simulink model "commqpsktxrx_18b"  (R2018b)
settings: Solver=FixedStepDiscrete  StartTime=0.0  StopTime=inf  RelTol=1e-3
PreLoadFcn:
  | qpsktxrx = commqpsktxrx_init();
InitFcn:
  | qpsktxrx = commqpsktxrx_init();
StopFcn:
  | if (strcmp(get_param([bdroot, '/Model Parameters'],'ShowRecvMsg'),'on'))
  |   if exist('Received','var')
  |      fprintf('%s', Received.signals.values);
  |   end
  | end
undefined symbols (not defined in the file or in its folder): Fs, ip, usb
libraries: dspsigops x3, commdigbbndpm3 x3, commsync2 x3, plutoradiolib x2, simulink x2, commrflib2 x2, commrfcorlib x2, dspstat3 x2, commutil2 x2, commsequence2 x2, dspsrcs4 x2, commfilt2 x2
Description:
  | QPSK Transmitter and Receiver.
  | 
  | This model shows the implementation of a QPSK transmitter and receiver.
settings Model: FPTRunName=Active  Creator=The MathWorks, Inc.  LastModifiedBy=KingSei
settings DataIOCC: LimitDataPoints=on  SaveFormat=Array  SaveOutput=off  SaveTime=off
settings OptimizationCC: BooleanDataType=off  DefaultParameterBehavior=Inlined  ExpressionDepthLimit=2147483647  LocalBlockOutputs=off  LifeSpan=inf
settings DebuggingCC: AlgebraicLoopMsg=error  UnderspecifiedInitializationDetection=Classic  MergeDetectMultiDrivingBlocksExec=none  SolverPrmCheckMsg=warning  SingleTaskRateTransMsg=error  ParameterPrecisionLossMsg=none  FcnCallInpInsideContextMsg=warning  AllowSymbolicDim=off  StateNameClashWarn=warning  SFUnexpectedBacktrackingDiag=warning  SFNoUnconditionalDefaultTransitionDiag=warning  SFExecutionAtInitializationDiag=none
settings HardwareCC: ProdBitPerPointer=32  ProdBitPerSizeT=32  ProdBitPerPtrDiffT=32  ProdLargestAtomicFloat=None  ProdIntDivRoundTo=Undefined  ProdEndianess=Unspecified  ProdWordSize=32  ProdHWDeviceType=32-bit Generic  TargetBitPerPointer=64  TargetBitPerSizeT=64  TargetBitPerPtrDiffT=64  TargetLongLongMode=on  TargetIntDivRoundTo=Zero  TargetEndianess=LittleEndian  TargetWordSize=64  TargetHWDeviceType=Generic->MATLAB Host Computer  ProdEqTarget=off
settings ModelReferenceCC: PropagateSignalLabelsOutOfModel=off
settings SFSimCC: SimUseLocalCustomCode=off
settings RTWCC: Description=Generic Real-Time Target  RTWUseLocalCustomCode=off
settings CodeAppCC: StateflowObjectComments=on
settings GRTTargetCC: TargetLangStandard=C89/C90 (ANSI)
settings ConfigComp: CovMetricSettings=dw  CovSaveCumulativeToWorkspaceVar=on  CovSaveSingleToWorkspaceVar=on  CovExternalEMLEnable=off  CovSFcnEnable=off

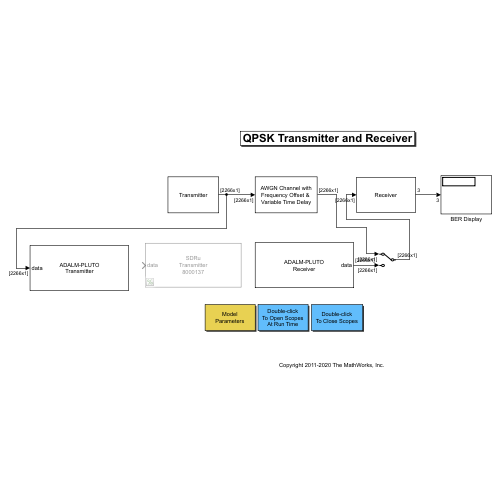
[thumbnail: Simulink's stored preview of the top-level diagram]
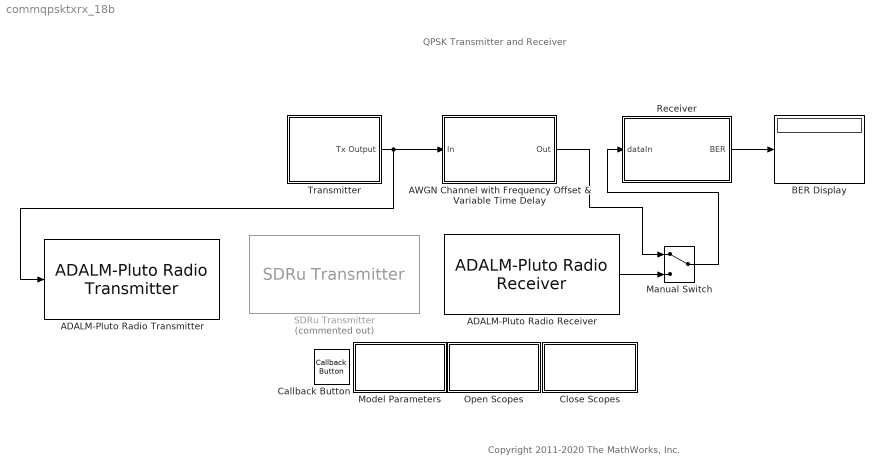
== system commqpsktxrx_18b ==
  note: QPSK Transmitter and Receiver
  note: Copyright 2011-2020 The MathWorks, Inc.
  ADALM-Pluto Radio Receiver : plutoradiolib/ADALM-Pluto Radio Receiver  RadioID=usb:0  uri=ip:10.0.0.200  CenterFrequencySource=Dialog  CenterFrequency=915e6-5e3  GainSource=AGC Slow Attack  GainSourceBlock=Dialog  Gain=50  ChannelMapping=1  BasebandSampleRate=1e5  OutputDataType=double  SamplesPerFrame=2266  OverflowOutputPort=off  EnableBurstMode=off  NumFramesInBurst=1  ShowAdvancedProperties=off  UseCustomFilter=off  filtPathRates=[737280000 11520000 3840000 1920000 960000 240000]  filtCoefficients=[-192 82 85 -215 228 -102 -110 290 -318 145 160 -426 471 -215 -238 633 -697 318 349 -923 1009 -457 -498 1309 -1423 640 693 -1812 1959 -876 -945 2458 -2647 1180 1268 -3290 3534 -1572 -1688 4375 -4698 2091 2247 -5836 6284 -2807 -3031 7918 -8588 3870 4225 -11182 12324 -5662 -6330 17255 -19735 9507 11312 -33568 43355 -25227 -42139 305542 305542 -42139 -25227 43355 -33568 11312 9507 -19735 17255 -6330 -5662 12324 -11182 4225 3870 -8588 7918 -3031 -2807 6284 -5836 2247 2091 -4698 4375 -1688 -1572 3534 -3290 1268 1180 -2647 2458 -945 -876 1959 -1812 693 640 -1423 1309 -498 -457 1009 -923 349 318 -697 633 -238 -215 471 -426 160 145 -318 290 -110 -102 228 -215 85 82 -192]  filtCoefficientSize=128  filtDecimInterpFactor=4  filtGain=-12  filtRFBandwidth=18000000  filterConfigStruct=struct()  EnableQuadratureCorrection=on  EnableRFDCCorrection=on  EnableBasebandDCCorrection=on  FrequencyCorrection=0  OverrideSampleTime=off  SampleTime=0.02  DataTimeout=Inf  ENSMPinControlMode=None  BISTLoopbackMode=Disabled  BISTToneInject=Disabled  BISTSignalGen=PRBS  BISTToneFreq=Fs/32  BISTToneLevel=0
  ADALM-Pluto Radio Transmitter : plutoradiolib/ADALM-Pluto Radio Transmitter  RadioID=usb:0  uri=ip:10.0.0.200  CenterFrequencySource=Dialog  CenterFrequency=915e6  GainSource=Dialog  Gain=-10  ChannelMapping=1  BasebandSampleRate=1e5  UnderflowOutputPort=off  ShowAdvancedProperties=off  UseCustomFilter=off  filtPathRates=[737280000 11520000 3840000 1920000 960000 240000]  filtCoefficients=[-192 82 85 -215 228 -102 -110 290 -318 145 160 -426 471 -215 -238 633 -697 318 349 -923 1009 -457 -498 1309 -1423 640 693 -1812 1959 -876 -945 2458 -2647 1180 1268 -3290 3534 -1572 -1688 4375 -4698 2091 2247 -5836 6284 -2807 -3031 7918 -8588 3870 4225 -11182 12324 -5662 -6330 17255 -19735 9507 11312 -33568 43355 -25227 -42139 305542 305542 -42139 -25227 43355 -33568 11312 9507 -19735 17255 -6330 -5662 12324 -11182 4225 3870 -8588 7918 -3031 -2807 6284 -5836 2247 2091 -4698 4375 -1688 -1572 3534 -3290 1268 1180 -2647 2458 -945 -876 1959 -1812 693 640 -1423 1309 -498 -457 1009 -923 349 318 -697 633 -238 -215 471 -426 160 145 -318 290 -110 -102 228 -215 85 82 -192]  filtCoefficientSize=128  filtDecimInterpFactor=4  filtGain=-12  filtRFBandwidth=18000000  filterConfigStruct=struct()  DataSourceSelect=Input Port  DDSTone1Freq=5e3  DDSTone2Freq=10e3  DDSTone1Scale=0.5  DDSTone2Scale=0.25  DataTimeout=Inf  FrequencyCorrection=0  ENSMPinControlMode=None  BISTLoopbackMode=Disabled  BISTToneInject=Disabled  BISTSignalGen=PRBS  BISTToneFreq=Fs/32  BISTToneLevel=0
  AWGN Channel with Frequency Offset & Variable Time Delay : Subsystem
      mask Display: disp('AWGN Channel with\nFrequency Offset & \nVariable Time Delay');
  BER Display : Display
  Callback Button : CallbackButton  WebBlockId=1825  PressDelay=500  RepeatInterval=0  ButtonText=?
      settings: ClickFcn=showExample('comm/QPSKTransmitterAndReceiverSimulinkExample')
  Close Scopes : Subsystem
      settings: OpenFcn=|
      | close_system([bdroot '/Receiver/Spectrum']);
      | set_param([bdroot '/Receiver/Spectrum'],'OpenScopeAtSimStart','off');
      | 
      | close_system([bdroot '/Receiver/After RC Rx Filter']);
      | set_param([bdroot '/Receiver/After RC Rx Filter'],'OpenScopeAtSimStart','off');
      | 
      | close_system([bdroot '/Receiver/After Carrier Synchronizer']);
      | set_param([bdroot '/Receiver/After Carrier Synchronizer'],'OpenScopeAtSimStart','off');
      | 
      | close_system([bdroot '/Receiver/After Symbol Synchronizer']);
      | set_param([bdroot '/Receiver/After Symbol Synchronizer'],'OpenScopeAtSimStart','off');
      mask Display: disp('Double-click\nTo Close Scopes');
  Manual Switch : ManualSwitch
  Model Parameters : Subsystem  mask(Model Parameters){SettingCtrl=Channel impairment settings, EbN0dB=20, FreqOffset=5e3, DelayCtrl=Triangle, DelayStep=0.0125*qpsktxrx.Interpolation, MinDelay=0, MaxDelay=2*qpsktxrx.Interpolation, DelayStart=0.1, CFCAlgorithm=Correlation-based, MaxOffset=6e3, FreqResolution=25, FineFreqNormalizedLoopBW=0.01, FineFreqDampingFactor=1, TimeRecNormalizedLoopBW=0.01, TimeRecDampingFactor=1, ShowRecvMsg=on}
      mask prompts: SettingCtrl "Setting types:"; EbN0dB "Eb/No (dB):"; FreqOffset "Frequency offset (Hz):"; DelayCtrl "Delay type:"; DelayStep "Delay step (samples/frame):"; MinDelay "Minimum delay (samples):"; MaxDelay "Maximum delay (samples):"; DelayStart "Start delay (samples):"; CFCAlgorithm "Algorithm:"; MaxOffset "Maximum frequency offset:"; FreqResolution "Desired frequency resolution (Hz):"; FineFreqNormalizedLoopBW "Normalized loop bandwidth:"; FineFreqDampingFactor "Damping factor:"; TimeRecNormalizedLoopBW "Normalized loop bandwidth:"; TimeRecDampingFactor "Damping factor:"; ShowRecvMsg "Show received message:"
      mask help: Choose to set the channel impairment parameters, parameters for the coarse frequency compensation, PLL parameters for fine frequency compensation and timing recovery.
      mask init:
      | myException = commqpsktxrx_mask(gcb, 'init', DelayCtrl, MinDelay,...
      |   MaxDelay, DelayStart, DelayStep);
      | if ~isempty(myException)
      |   errordlg(myException.msg);
      | end
      mask Help: helpview(commdhelp);
      mask TypeOptions SettingCtrl: Channel impairment settings | Coarse frequency compensation settings | Fine frequency compensation settings | Timing recovery settings
      mask Callback SettingCtrl: commqpsktxrx_mask(gcbh, 'cbShowHideSettingOptions');
      mask TypeOptions DelayCtrl: Ramp | Triangle
      mask Callback DelayCtrl: commqpsktxrx_mask(gcbh, 'cbShowHideDelayOptions');
      mask TypeOptions CFCAlgorithm: Correlation-based | FFT-based
      mask Callback CFCAlgorithm: commqpsktxrx_mask(gcbh, 'cbShowHideCFCOptions');
      mask Display: disp('Model\nParameters');
  Open Scopes : Subsystem
      settings: OpenFcn=|
      | open_system([bdroot '/Receiver/Spectrum']);
      | set_param([bdroot '/Receiver/Spectrum'],'OpenScopeAtSimStart','on');
      | 
      | open_system([bdroot '/Receiver/After RC Rx Filter']);
      | set_param([bdroot '/Receiver/After RC Rx Filter'],'OpenScopeAtSimStart','on');
      | 
      | open_system([bdroot '/Receiver/After Carrier Synchronizer']);
      | set_param([bdroot '/Receiver/After Carrier Synchronizer'],'OpenScopeAtSimStart','on');
      | 
      | open_system([bdroot '/Receiver/After Symbol Synchronizer']);
      | set_param([bdroot '/Receiver/After Symbol Synchronizer'],'OpenScopeAtSimStart','on');
      mask Display: disp('Double-click\nTo Open Scopes\nAt Run Time');
  Receiver : Subsystem
      mask Display: disp('Receiver')
  SDRu Transmitter : commsdrhw_v2/SDRu Transmitter  Commented=on  rxtx=tx  initializeIPAddress=0  devMap=0  USRP2_IP=192.168.10.2  USRP_IP_X300=192.168.10.2  USRP_IP_X310=192.168.10.2  USRP_IP_N300=No devices found  USRP_IP_N310=192.168.10.2  USRP_IP_N320=No devices found  USRP_serialNumB200=No devices found  USRP_serialNumB210=8000137  platform=B210  prevPlatform=B210  lastIPAddressPopup=192.168.10.2  USRP_ID=8000137  LastIPAddress=192.168.10.2  ChannelMapping=1  centerFrequencySrc=Dialog  centerFrequency=915e6  loOffsetSrc=Dialog  loOffset=0  gainSrc=Dialog  gain=30  PPSSource=Internal  EnableGPSLock=off  EnsureSyncGPSTime=off  clockSource=Internal  EnableRefLock=off  masterClkRateParam=32000000  masterClkRateB200=32e6  masterClkRateB210=32e6  masterClkRateX300=200e6  masterClkRateX310=200e6  masterClkRateN300=125e6  masterClkRateN310=125e6  masterClkRateN320=200e6  decimInterpSrc=Dialog  lastDecimSource=Dialog  decimInterp=320  USRP2_IP_NUM=[56 48 48 48 49 51 55]  frameLength=362  sampleRate=100000  TransportDataType=int16  outputDatatype=Same as transport data type  overrunUnderrunPort=off  sampleTime=5.12e-06  dboardInfo=|  HOST_DATA_PORT=30000  HOST_CONTROL_PORT=30001  USRP2_DATA_PORT=32769  USRP2_CONTROL_PORT=32768  bufferMode=Continuous streaming  EnableBurstMode=off  NumFramesInBurst=100
      | dbid: 0
      |           dbName: 'no db found'
      |          freqMin: 0
      |          freqMax: 0
      |          gainMin: 0
      |          gainMax: 0
      |     gainStepSize: 0
  Transmitter : Subsystem
      mask Display: disp('Transmitter')
  wires:
  Transmitter/1(Tx Output) -> ADALM-Pluto Radio Transmitter/1, AWGN Channel with Frequency Offset & Variable Time Delay/1(In)
  Receiver/1(BER) -> BER Display/1
  ADALM-Pluto Radio Receiver/1 -> Manual Switch/2
  AWGN Channel with Frequency Offset & Variable Time Delay/1(Out) -> Manual Switch/1
  Manual Switch/1 -> Receiver/1(dataIn)

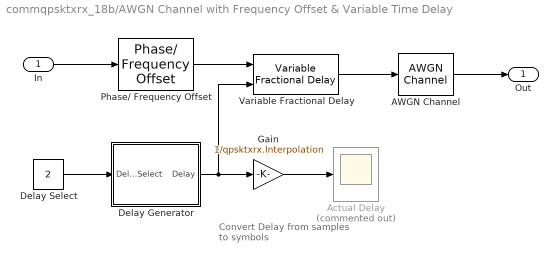
== system commqpsktxrx_18b/AWGN Channel with Frequency Offset & Variable Time Delay ==
  note: Convert Delay from
      | samples to symbols
  In : Inport
  AWGN Channel : commchan3/AWGN Channel  InputProcessing=Columns as channels (frame based)  noiseMode="Signal to noise ratio  (Eb/No)"  EbNodB=20  EsNodB=15  SNRdB=15  bitsPerSym=log2(qpsktxrx.ModulationOrder)  Ps=1/qpsktxrx.Interpolation  Tsym=qpsktxrx.Tsym  variance=1  seed=2
  Actual Delay : Scope  Commented=on
  Delay Generator : Subsystem
      mask Display: disp('Delay Generator')
  Delay Select : Constant  Value=2
  Gain : Gain  Gain=1/qpsktxrx.Interpolation
  Phase/ Frequency Offset : commrflib2/Phase// Frequency Offset  phaseOffset=qpsktxrx.PhaseOffset  freqPort=off  freqOffset=5000
  Variable Fractional Delay : dspsigops/Variable Fractional Delay  mode=OBSOLETE  modeActive=Linear  L=4  FarrowL=4  R=10  alpha=1  dmax=qpsktxrx.FrameSize*qpsktxrx.Interpolation  InputProcessing=Columns as channels (frame based)  ic=0  noDFT=off  fallbackFIR=Clip to the minimum value necessary for centered kernel  fallbackFarrow=Clip to the minimum value necessary for centered kernel  roundingMode=Zero  overflowMode=off
  Out : Outport  VectorParamsAs1DForOutWhenUnconnected=off
  wires:
  AWGN Channel/1 -> Out/1
  In/1 -> Phase/ Frequency Offset/1
  Phase/ Frequency Offset/1 -> Variable Fractional Delay/1
  Variable Fractional Delay/1 -> AWGN Channel/1
  Delay Select/1 -> Delay Generator/1(Delay Select)
  Delay Generator/1(Delay) -> Variable Fractional Delay/2, Gain/1
  Gain/1 -> Actual Delay/1

== system commqpsktxrx_18b/Close Scopes ==

== system commqpsktxrx_18b/Model Parameters ==

== system commqpsktxrx_18b/Open Scopes ==

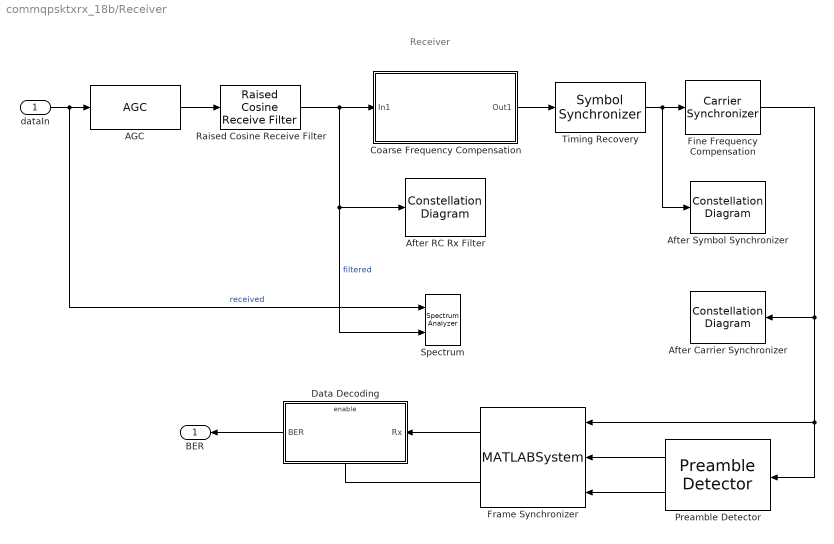
== system commqpsktxrx_18b/Receiver ==
  note: Receiver
  dataIn : Inport
  AGC : commrfcorlib/AGC  LegacyMode=off  DetectorMethod=Rectifier  LoopMethod=Linear  UpdatePeriod=100  StepSize=0.1  AdaptationStepSize=0.01  DesiredOutputPower=qpsktxrx.DesiredPower  AveragingLength=qpsktxrx.AveragingLength  MaximumGain=30  MaxPowerGain=qpsktxrx.MaxPowerGain  GainOutputPort=off  InputPowerOutputPort=off  SimulateUsing=Code generation
  After Carrier Synchronizer : ConstellationDiagram  Tag=ScatterPlot  DefaultConfigurationName=comm.scopes.ConstellationDiagramBlockCfg
  After RC Rx Filter : ConstellationDiagram  Tag=ScatterPlot  DefaultConfigurationName=comm.scopes.ConstellationDiagramBlockCfg
  After Symbol Synchronizer : ConstellationDiagram  Tag=ScatterPlot  DefaultConfigurationName=comm.scopes.ConstellationDiagramBlockCfg
  Coarse Frequency Compensation : Subsystem
      mask Display: fprintf('Coarse Frequency\nCompensation')
  Data Decoding : Subsystem
      mask Display: disp('Data Decoding');
  Fine Frequency Compensation : commsync2/Carrier Synchronizer  Modulation=QPSK  ModulationPhaseOffset=Auto  CustomPhaseOffset=0  SamplesPerSymbol=qpsktxrx.Interpolation/qpsktxrx.Decimation  DampingFactor=1  NormalizedLoopBandwidth=0.01  EstimatedPhaseErrorOutputPort=off  SimulateUsing=Code generation
  Frame Synchronizer : MATLABSystem  System=FrameSynchronizer  Input=Symbol  OutputFrameLength=qpsktxrx.FrameSize  PreambleLength=qpsktxrx.BarkerLength  SimulateUsing=Code generation
      mask Type: FrameSynchronizer
      mask Display:
      | disp(['Frame' char(10) 'Synchronizer']);
      | port_label('input',1,'u');
      | port_label('input',2,'idx');
      | port_label('input',3,'dtMt');
      | port_label('output',1,'Frame');
      | port_label('output',2,'Valid');
  Preamble Detector : commsync2/Preamble Detector  Input=Symbol  Preamble=sqrt(2)/2 * (-1-1i) * (qpsktxrx.BarkerCode)'  Threshold=qpsktxrx.PreambleDetectorThreshold  DetectionMetricOutput=on  Detections=All  SimulateUsing=Code generation
  Raised Cosine Receive Filter : commfilt2/Raised Cosine Receive Filter  filtType=Square root  R=qpsktxrx.RolloffFactor  filtSpan=qpsktxrx.RaisedCosineFilterSpan  N=qpsktxrx.Interpolation  downFactor=qpsktxrx.Decimation  downOffset=0  filterGain=1  InputProcessing=Columns as channels (frame based)  RateOptions=Enforce single-rate processing  framing=Mute  checkCoeff=off  variableName=rcRxFilt  currentFiltSpan=10  D=5  inputOffset=0  sampMode=Mute  saveAsFlag=0  rateMode=Downsampling  checkGain=Normalized  launchFVT=on  roundingMode=Floor  overflowMode=off  coeffDataTypeStr=Inherit: Same word length as input  coeffMin=[]  coeffMax=[]  coeffLastDataTypeStr=Inherit: Same word length as input  accumDataTypeStr=Inherit: Same as product output  accumLastDataTypeStr=Inherit: Same as product output  outputDataTypeStr=Inherit: Same as accumulator  outputMin=[]  outputMax=[]  outputLastDataTypeStr=Inherit: Same as accumulator
  Spectrum : SpectrumAnalyzer  NumInputPorts=2  DefaultConfigurationName=spbscopes.SpectrumAnalyzerBlockCfg
  Timing Recovery : commsync2/Symbol Synchronizer  Modulation=PAM/PSK/QAM  TimingErrorDetector=Gardner (non-data-aided)  SamplesPerSymbol=qpsktxrx.Interpolation/qpsktxrx.Decimation  DampingFactor=1  NormalizedLoopBandwidth=0.01  DetectorGain=qpsktxrx.TimingErrorDetectorGain  TimingErrorOutputPort=off  SimulateUsing=Code generation
  BER : Outport  VectorParamsAs1DForOutWhenUnconnected=off
  wires:
  Raised Cosine Receive Filter/1 -> Coarse Frequency Compensation/1(In1), Spectrum/2, After RC Rx Filter/1  "filtered"
  dataIn/1 -> Spectrum/1, AGC/1  "received"
  AGC/1 -> Raised Cosine Receive Filter/1
  Timing Recovery/1 -> Fine Frequency Compensation/1, After Symbol Synchronizer/1
  Coarse Frequency Compensation/1(Out1) -> Timing Recovery/1
  Fine Frequency Compensation/1 -> Frame Synchronizer/1, Preamble Detector/1, After Carrier Synchronizer/1
  Frame Synchronizer/1 -> Data Decoding/1(Rx)
  Preamble Detector/1 -> Frame Synchronizer/2
  Preamble Detector/2 -> Frame Synchronizer/3
  Frame Synchronizer/2 -> Data Decoding/Enable
  Data Decoding/1(BER) -> BER/1

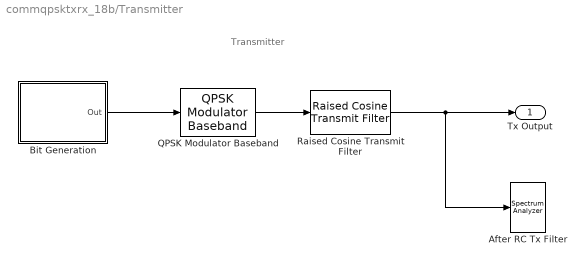
== system commqpsktxrx_18b/Transmitter ==
  note: Transmitter
  After RC Tx Filter : SpectrumAnalyzer  DefaultConfigurationName=spbscopes.SpectrumAnalyzerBlockCfg
  Bit Generation : Subsystem
      mask Display: disp('Bits Generation')
  QPSK Modulator Baseband : commdigbbndpm3/QPSK Modulator Baseband  InType=Bit  Enc=Gray  Ph=pi/4  outDtype=double  outWordLen=16  outUDDataType=sfix(16)  outFracLenMode=Best precision  outFracLen=15  outDataTypeStr=double  outLastDataTypeStr=double
  Raised Cosine Transmit Filter : commfilt2/Raised Cosine Transmit Filter  filtType=Square root  R=qpsktxrx.RolloffFactor  filtSpan=qpsktxrx.RaisedCosineFilterSpan  N=qpsktxrx.Interpolation  filterGain=1  InputProcessing=Columns as channels (frame based)  RateOptions=Enforce single-rate processing  framing=Mute  checkCoeff=off  variableName=rcTxFilt1  checkGain=Normalized  sampMode=Mute  saveAsFlag=0  currentFiltSpan=10  D=5  launchFVT=on  roundingMode=Floor  overflowMode=off  coeffDataTypeStr=Inherit: Same word length as input  coeffMin=[]  coeffMax=[]  coeffLastDataTypeStr=Inherit: Same word length as input  outputDataTypeStr=Inherit: Same as accumulator  outputMin=[]  outputMax=[]  outputLastDataTypeStr=Inherit: Same as accumulator
  Tx Output : Outport  VectorParamsAs1DForOutWhenUnconnected=off
  wires:
  QPSK Modulator Baseband/1 -> Raised Cosine Transmit Filter/1
  Raised Cosine Transmit Filter/1 -> Tx Output/1, After RC Tx Filter/1
  Bit Generation/1(Out) -> QPSK Modulator Baseband/1

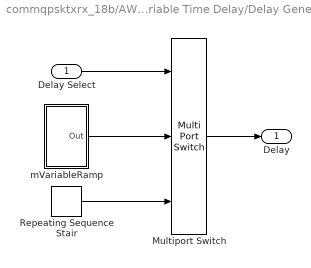
== system commqpsktxrx_18b/AWGN Channel with Frequency Offset & Variable Time Delay/Delay Generator ==
  Delay Select : Inport
  Multiport Switch : MultiPortSwitch  Inputs=2  OutDataTypeStr=double
  Repeating Sequence Stair : simulink/Sources/Repeating Sequence Stair  OutValues="[0       0.025        0.05       0.075         0.1       0.125        0.15       0.175         0.2       0.225        0.25       0.275         0.3       0.325        0.35       0.375         0.4       0.425        0.45       0.475         0.5       0.525        0.55       0.575         0.6       0.625        0.65       0.675         0.7       0.725        0.75       0.775         0.8       0.825        0.85       0.875         0.9       0.925        0.95       0.975           1       1.025        1.05       1.075         1.1       1.125        1.15       1.175         1.2       1.225        1.25       1.275         1.3       1.325        1.35       1.375         1.4       1.425        1.45       1.475         1.5       1.525        1.55       1.575         1.6       1.625        1.65       1.675         1.7       1.725        1.75       1.775         1.8       1.825        1.85       1.875         1.9       1.925        1.95       1.975           2       2.025        2.05       2.075         2.1       2.125        2.15       2.175         2.2       2.225        2.25       2.275         2.3       2.325        2.35       2.375         2.4       2.425        2.45       2.475         2.5       2.525        2.55       2.575         2.6       2.625        2.65       2.675         2.7       2.725        2.75       2.775         2.8       2.825        2.85       2.875         2.9       2.925        2.95       2.975           3       3.025        3.05       3.075         3.1       3.125        3.15       3.175         3.2       3.225        3.25       3.275         3.3       3.325        3.35       3.375         3.4       3.425        3.45       3.475         3.5       3.525        3.55       3.575         3.6       3.625        3.65       3.675         3.7       3.725        3.75       3.775         3.8       3.825        3.85       3.875         3.9       3.925        3.95       3.975           4       3.975        3.95       3.925         3.9       3.875        3.85       3.825         3.8       3.775        3.75       3.725         3.7       3.675        3.65       3.625         3.6       3.575        3.55       3.525         3.5       3.475        3.45       3.425         3.4       3.375        3.35       3.325         3.3       3.275        3.25       3.225         3.2       3.175        3.15       3.125         3.1       3.075        3.05       3.025           3       2.975        2.95       2.925         2.9       2.875        2.85       2.825         2.8       2.775        2.75       2.725         2.7       2.675        2.65       2.625         2.6       2.575        2.55       2.525         2.5       2.475        2.45       2.425         2.4       2.375        2.35       2.325         2.3       2.275        2.25       2.225         2.2       2.175        2.15       2.125         2.1       2.075        2.05       2.025           2       1.975        1.95       1.925         1.9       1.875        1.85       1.825         1.8       1.775        1.75       1.725         1.7       1.675        1.65       1.625         1.6       1.575        1.55       1.525         1.5       1.475        1.45       1.425         1.4       1.375        1.35       1.325         1.3       1.275        1.25       1.225         1.2       1.175        1.15       1.125         1.1       1.075        1.05       1.025           1       0.975        0.95       0.925         0.9       0.875        0.85       0.825         0.8       0.775        0.75       0.725         0.7       0.675        0.65       0.625         0.6       0.575        0.55       0.525         0.5       0.475        0.45       0.425         0.4       0.375        0.35       0.325         0.3       0.275        0.25       0.225         0.2       0.175        0.15       0.125         0.1       0.075        0.05       0.025]"  tsamp=qpsktxrx.FrameTime  OutMin=[]  OutMax=[]  OutDataTypeStr=double  OutputDataTypeScalingMode=double  OutDataType=fixdt(0,8)  ConRadixGroup=Best Precision: Vector-wise  OutScaling=2^-12
  mVariableRamp : Subsystem
  Delay : Outport  VectorParamsAs1DForOutWhenUnconnected=off
  wires:
  Delay Select/1 -> Multiport Switch/1
  Repeating Sequence Stair/1 -> Multiport Switch/3
  mVariableRamp/1(Out) -> Multiport Switch/2
  Multiport Switch/1 -> Delay/1

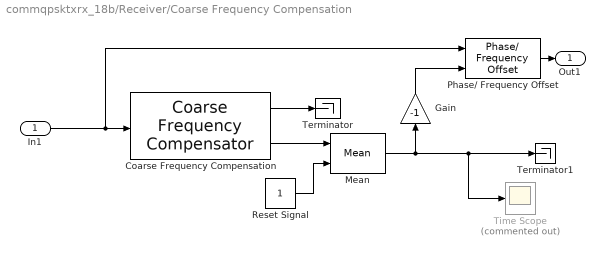
== system commqpsktxrx_18b/Receiver/Coarse Frequency Compensation ==
  In1 : Inport
  Coarse Frequency Compensation : commrfcorlib/Coarse Frequency Compensator  Modulation=QPSK  Algorithm=Correlation-based  FrequencyResolution=25  MaximumFrequencyOffset=6000  SamplesPerSymbol=4  EstimatedFreqOffsetPort=on  SimulateUsing=Code generation
  Gain : Gain  Gain=-1
  Mean : dspstat3/Mean  run=on  InputProcessing=Columns as channels (frame based)  reset_popup=Either edge  directionMode=Each column  dimension=1  roiEnable=off  roiType=Rectangles  roiPortion=Entire ROI  roiOutput=Individual statistics for each ROI  roiFlag=off  roundingMode=Floor  overflowMode=off  outputDataTypeStr=Inherit: Same as accumulator  outputMin=[]  outputMax=[]  outputLastDataTypeStr=Inherit: Same as accumulator
  Phase/ Frequency Offset : commrflib2/Phase// Frequency Offset  phaseOffset=0  freqPort=on  freqOffset=0
  Reset Signal : Constant
  Terminator : Terminator
  Terminator1 : Terminator
  Time Scope : Scope  Commented=on
  Out1 : Outport  VectorParamsAs1DForOutWhenUnconnected=off
  wires:
  In1/1 -> Phase/ Frequency Offset/1, Coarse Frequency Compensation/1
  Phase/ Frequency Offset/1 -> Out1/1
  Mean/1 -> Time Scope/1, Terminator1/1, Gain/1
  Coarse Frequency Compensation/2 -> Mean/1
  Coarse Frequency Compensation/1 -> Terminator/1
  Gain/1 -> Phase/ Frequency Offset/2
  Reset Signal/1 -> Mean/2

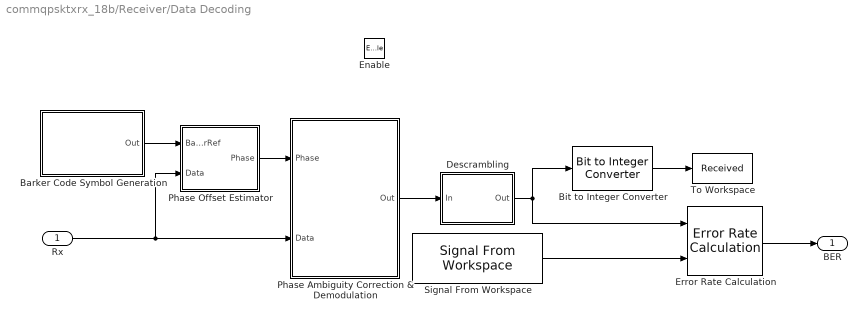
== system commqpsktxrx_18b/Receiver/Data Decoding ==
  Rx : Inport
  Enable : EnablePort
  "Barker Code Symbol Generation " : Subsystem
      mask Display: disp('Barker Code\nSymbol Generation')
  Bit to Integer Converter : commutil2/Bit to Integer Converter  nbits=7  bitOrder=MSB first  signedOutputValues=Unsigned  outDtype=Inherit via internal rule  outDtypeSigned=Inherit via internal rule
  Descrambling : Subsystem
      mask Display: disp('Descrambling');
  Error Rate Calculation : commsink2/Error Rate Calculation  N=0  st_delay=0  cp_mode=Select samples from mask  subframe=qpsktxrx.BerMask  PMode=Port  WsName=ErrorVec  RsMode2=off  stop=off  numErr=100  maxBits=1e6
  Phase Ambiguity Correction & Demodulation : Subsystem
      mask Display: disp('Phase Ambiguity\nCorrection\n& Demodulation');
  Phase Offset Estimator : Subsystem
  Signal From Workspace : dspsrcs4/Signal From Workspace  X=qpsktxrx.MessageBits  Ts=1/qpsktxrx.PayloadLength*qpsktxrx.FrameTime  nsamps=qpsktxrx.MessageLength * 7 * qpsktxrx.NumberOfMessage  OutputAfterFinalValue=Cyclic repetition  ignoreOrWarnInputAndFrameLengths=off  OutputFrames=off
  To Workspace : ToWorkspace  VariableName=Received  SaveFormat=Structure  SampleTime=-1
      settings: Save2DSignal=2-D array (concatenate along first dimension)
  BER : Outport  VectorParamsAs1DForOutWhenUnconnected=off
  wires:
  "Barker Code Symbol Generation "/1(Out) -> Phase Offset Estimator/1(BarkerRef)
  Phase Offset Estimator/1(Phase) -> Phase Ambiguity Correction & Demodulation/1(Phase)
  Rx/1 -> Phase Offset Estimator/2(Data), Phase Ambiguity Correction & Demodulation/2(Data)
  Descrambling/1(Out) -> Error Rate Calculation/1, Bit to Integer Converter/1
  Error Rate Calculation/1 -> BER/1
  Phase Ambiguity Correction & Demodulation/1(Out) -> Descrambling/1(In)
  Signal From Workspace/1 -> Error Rate Calculation/2
  Bit to Integer Converter/1 -> To Workspace/1

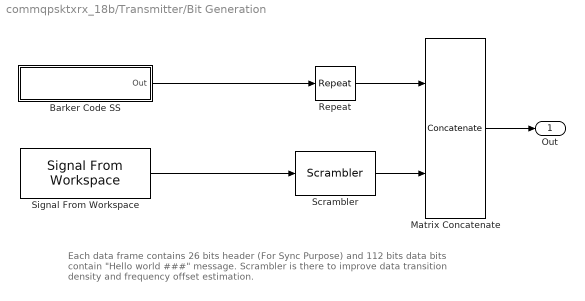
== system commqpsktxrx_18b/Transmitter/Bit Generation ==
  note: Each data frame contains 26 bits header (For Sync Purpose) and 112 bits data bits
      | contain "Hello world ###" message. Scrambler is there to improve data
      | transition density and frequency offset estimation.
  Barker Code SS : Subsystem
      mask Display: disp('Unipolar\nBarker Code')
  Matrix Concatenate : Concatenate  Mode=Multidimensional array
  Repeat : dspsigops/Repeat  N=2  InputProcessing=Columns as channels (frame based)  RateOptions=Enforce single-rate processing  ic=0  mode=Unused parameter value
  Scrambler : commsequence2/Scrambler  M=2  poly=[1 1 1 0 1]  iniStaSource=Dialog Parameter  ini_sta=[0 0 0 0]  resetViaPort=off
  Signal From Workspace : dspsrcs4/Signal From Workspace  X=qpsktxrx.MessageBits  Ts=1/qpsktxrx.PayloadLength*qpsktxrx.FrameTime  nsamps=qpsktxrx.MessageLength * 7 * qpsktxrx.NumberOfMessage  OutputAfterFinalValue=Cyclic repetition  ignoreOrWarnInputAndFrameLengths=off  OutputFrames=off
  Out : Outport  VectorParamsAs1DForOutWhenUnconnected=off
  wires:
  Barker Code SS/1(Out) -> Repeat/1
  Matrix Concatenate/1 -> Out/1
  Repeat/1 -> Matrix Concatenate/1
  Scrambler/1 -> Matrix Concatenate/2
  Signal From Workspace/1 -> Scrambler/1

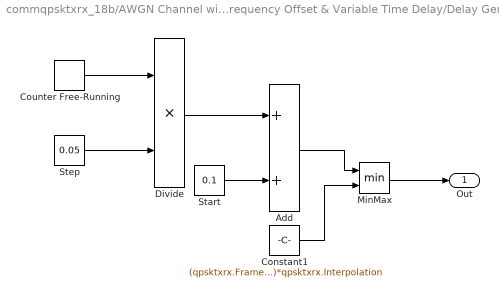
== system commqpsktxrx_18b/AWGN Channel with Frequency Offset & Variable Time Delay/Delay Generator/mVariableRamp ==
  Add : Sum
  Constant1 : Constant  Value=(qpsktxrx.FrameSize-qpsktxrx.RaisedCosineFilterSpan)*qpsktxrx.Interpolation
  Counter Free-Running : simulink/Sources/Counter Free-Running  NumBits=64  tsamp=qpsktxrx.FrameTime
  Divide : Product  Inputs=**
  MinMax : MinMax  Inputs=2
  Start : Constant  Value=0.1
  Step : Constant  Value=0.05
  Out : Outport  VectorParamsAs1DForOutWhenUnconnected=off
  wires:
  Counter Free-Running/1 -> Divide/1
  Step/1 -> Divide/2
  Divide/1 -> Add/1
  Start/1 -> Add/2
  Add/1 -> MinMax/1
  MinMax/1 -> Out/1
  Constant1/1 -> MinMax/2

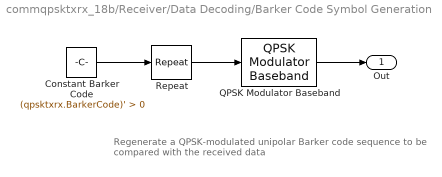
== system commqpsktxrx_18b/Receiver/Data Decoding/Barker Code Symbol Generation  ==
  note: Regenerate a QPSK-modulated unipolar Barker code sequence
      | to be compared with the received data
  Constant Barker Code : Constant  Value=(qpsktxrx.BarkerCode)' > 0  VectorParams1D=off  OutDataTypeStr=double
  QPSK Modulator Baseband : commdigbbndpm3/QPSK Modulator Baseband  InType=Bit  Enc=Gray  Ph=pi/4  outDtype=double  outWordLen=16  outUDDataType=sfix(16)  outFracLenMode=Best precision  outFracLen=15  outDataTypeStr=double  outLastDataTypeStr=double
  Repeat : dspsigops/Repeat  N=2  InputProcessing=Columns as channels (frame based)  RateOptions=Enforce single-rate processing  ic=0  mode=Unused parameter value
  Out : Outport  VectorParamsAs1DForOutWhenUnconnected=off
  wires:
  Constant Barker Code/1 -> Repeat/1
  Repeat/1 -> QPSK Modulator Baseband/1
  QPSK Modulator Baseband/1 -> Out/1

== system commqpsktxrx_18b/Receiver/Data Decoding/Descrambling ==
  In : Inport
  Descrambler : commsequence2/Descrambler  M=2  poly=[1 1 1 0 1]  iniStaSource=Dialog Parameter  ini_sta=[0 0 0 0]  resetViaPort=off
  Selector : Selector  IndexOptions=Index vector (dialog)  Indices=[qpsktxrx.HeaderLength+(1 : qpsktxrx.PayloadLength)]  OutputSizes=1
  Out : Outport  VectorParamsAs1DForOutWhenUnconnected=off
  wires:
  In/1 -> Selector/1
  Selector/1 -> Descrambler/1
  Descrambler/1 -> Out/1

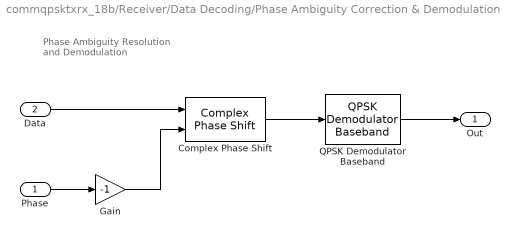
== system commqpsktxrx_18b/Receiver/Data Decoding/Phase Ambiguity Correction & Demodulation ==
  note: Phase Ambiguity Resolution
      | and Demodulation
  Phase : Inport
  Data : Inport  Port=2
  Complex Phase Shift : commutil2/Complex Phase Shift
  Gain : Gain  Gain=-1  OutDataTypeStr=Inherit: Same as input
  QPSK Demodulator Baseband : commdigbbndpm3/QPSK Demodulator Baseband  OutType=Bit  DecType=Hard decision  VarSource=Dialog  Variance=1  Dec=Gray  Ph=pi/4  outDtype1=Inherit via internal rule  outDtype2=Inherit via internal rule  derotateFactorWordLen=16  derotateFactorDataTypeStr=Inherit: Same word length as input  derotateFactorLastDataTypeStr=Inherit: Same word length as input
  Out : Outport  VectorParamsAs1DForOutWhenUnconnected=off
  wires:
  Phase/1 -> Gain/1
  Data/1 -> Complex Phase Shift/1
  Complex Phase Shift/1 -> QPSK Demodulator Baseband/1
  QPSK Demodulator Baseband/1 -> Out/1
  Gain/1 -> Complex Phase Shift/2

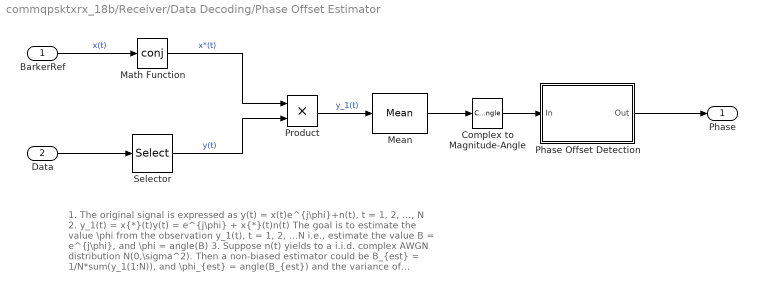
== system commqpsktxrx_18b/Receiver/Data Decoding/Phase Offset Estimator ==
  note: 1. The original signal is expressed as y(t) = x(t)e^{j\phi}+n(t), t = 1, 2, ..., N
      | 2. y_1(t) = x{*}(t)y(t) = e^{j\phi} + x{*}(t)n(t)
      | The goal is to estimate the value \phi from the observation y_1(t), t = 1, 2, ...N
      | i.e., estimate the value B = e^{j\phi}, and \phi = angle(B)
      | 3. Suppose n(t) yields to a i.i.d. complex AWGN distribution N(0,\sigma^2).
      | Then a non-biased estimator could be
      | B_{est} = 1/N*sum(y_1(1:N)), and \phi_{est} = angle(B_{est})
      | and the variance of B_{est} is \sigma^2/N
  BarkerRef : Inport
  Data : Inport  Port=2
  Complex to Magnitude-Angle : ComplexToMagnitudeAngle  Output=Angle
  Math Function : Math  Operator=conj  SaturateOnIntegerOverflow=on
  Mean : dspstat3/Mean  run=off  InputProcessing=Columns as channels (frame based)  reset_popup=None  directionMode=Each column  dimension=1  roiEnable=off  roiType=Rectangles  roiPortion=Entire ROI  roiOutput=Individual statistics for each ROI  roiFlag=off  roundingMode=Floor  overflowMode=off  outputDataTypeStr=Inherit: Same as accumulator  outputMin=[]  outputMax=[]  outputLastDataTypeStr=Inherit: Same as accumulator
  Phase Offset Detection : MATLAB Function  TreatAsAtomicUnit=on
  Product : Product  RndMeth=Zero
  Selector : Selector  IndexOptions=Index vector (dialog)  Indices=[1:qpsktxrx.BarkerLength]  OutputSizes=1
  Phase : Outport  VectorParamsAs1DForOutWhenUnconnected=off
  wires:
  Data/1 -> Selector/1
  BarkerRef/1 -> Math Function/1  "x(t)"
  Selector/1 -> Product/2  "y(t)"
  Math Function/1 -> Product/1  "x*(t)"
  Product/1 -> Mean/1  "y_1(t)"
  Mean/1 -> Complex to Magnitude-Angle/1
  Complex to Magnitude-Angle/1 -> Phase Offset Detection/1(In)
  Phase Offset Detection/1(Out) -> Phase/1

== system commqpsktxrx_18b/Transmitter/Bit Generation/Barker Code SS ==
  Constant Barker Code : Constant  Value=(qpsktxrx.BarkerCode)' > 0; % Bipolar to Unipolar  VectorParams1D=off  OutDataTypeStr=double
  Out : Outport  VectorParamsAs1DForOutWhenUnconnected=off
  wires:
  Constant Barker Code/1 -> Out/1

== matlab function commqpsktxrx_18b/Receiver/Data Decoding/Phase Offset Estimator/Phase Offset Detection ==
  data: In input; Out output
function Out = phasedecision(In)
% Map the estimated phase to one of -pi, -pi/2, 0, pi/2,  
%#codegen
Out = round(In.*2./pi)./2.*pi;
% The above processing is equivalent to the following processing using
% if/else statements
%
% if In<pi/4 && In>-pi/4
%     Out = 0;
% elseif In>=pi/4 && In<pi*3/4
%     Out = pi/2;
% elseif In>=pi*3/4 || In<=-pi*3/4
%     Out = -pi;
% else
%     Out = -pi/2;
% end
